simulink model "cable_driven_parallel_robot2022"  (R2022b)
settings: Solver=ode3  StartTime=0.0  StopTime=100  FixedStep=0.01  RelTol=1e-3
values from neighbouring files (symbols this model uses):
  cable_length = 1.2    [Model_Info.m]
  g = 9.81    [Model_Info.m]
  MP_H = 2    [Model_Info.m]
  MP_init_X = 0    [Model_Info.m]
  MP_init_Y = 0    [Model_Info.m]
  MP_init_Z = cable_length + (MP_H/2)    (= 2.2)    [Model_Info.m]
  MP_Ix = (MP_m/12)*(MP_W^2+MP_H^2)    (= 6.66666666667e-05)    [Model_Info.m]
  MP_Iy = (MP_m/12)*(MP_L^2+MP_H^2)    (= 6.66666666667e-05)    [Model_Info.m]
  MP_Iz = (MP_m/12)*(MP_L^2+MP_W^2)    (= 6.66666666667e-05)    [Model_Info.m]
  MP_L = 2    [Model_Info.m]
  MP_m = 0.0001    [Model_Info.m]
  MP_W = 2    [Model_Info.m]
  MR_init_X_L1 = -(MP_L/2)    (= -1)    [Model_Info.m]
  MR_init_X_L2 = (MP_L/2)    (= 1)    [Model_Info.m]
  MR_init_X_L3 = (MP_L/2)    (= 1)    [Model_Info.m]
  MR_init_X_L4 = -(MP_L/2)    (= -1)    [Model_Info.m]
  MR_init_Y_L1 = -(MP_W/2)    (= -1)    [Model_Info.m]
  MR_init_Y_L2 = -(MP_W/2)    (= -1)    [Model_Info.m]
  MR_init_Y_L3 = (MP_W/2)    (= 1)    [Model_Info.m]
  MR_init_Y_L4 = (MP_W/2)    (= 1)    [Model_Info.m]
  MR_init_Yaw_L1 = pi    (= 3.14159265359)    [Model_Info.m]
  MR_init_Yaw_L2 = 0    [Model_Info.m]
  MR_init_Yaw_L3 = 0    [Model_Info.m]
  MR_init_Yaw_L4 = pi    (= 3.14159265359)    [Model_Info.m]
  MR_Jr = (MR_m/12)*(MR_L^2+MR_W^2)    (= 0.333333333333)    [Model_Info.m]
  MR_m = 0.5    [Model_Info.m]
  MR_r = 2    [Model_Info.m]
  MR_WT = 2    [Model_Info.m]
  QR_Ax = 0.25*0    (= 0)    [Model_Info.m]
  QR_Ay = 0.25*0    (= 0)    [Model_Info.m]
  QR_Az = 0.25*0    (= 0)    [Model_Info.m]
  QR_b = 1.14*1e-7    (= 1.14e-07)    [Model_Info.m]
  QR_Ixx = 4.856*1e-3    (= 0.004856)    [Model_Info.m]
  QR_Iyy = 4.856*1e-3    (= 0.004856)    [Model_Info.m]
  QR_Izz = 8.801*1e-3    (= 0.008801)    [Model_Info.m]
  QR_K = 2.980*1e-6    (= 2.98e-06)    [Model_Info.m]
  QR_l = 0.225    [Model_Info.m]
  QR_m = 0.468    [Model_Info.m]
  QR_x0_U1 = -(MP_L/2)    (= -1)    [Model_Info.m]
  QR_x0_U2 = (MP_L/2)    (= 1)    [Model_Info.m]
  QR_x0_U3 = (MP_L/2)    (= 1)    [Model_Info.m]
  QR_x0_U4 = -(MP_L/2)    (= -1)    [Model_Info.m]
  QR_y0_U1 = -(MP_W/2)    (= -1)    [Model_Info.m]
  QR_y0_U2 = -(MP_W/2)    (= -1)    [Model_Info.m]
  QR_y0_U3 = (MP_W/2)    (= 1)    [Model_Info.m]
  QR_y0_U4 = (MP_W/2)    (= 1)    [Model_Info.m]
  QR_z0_U1 = 2*cable_length+(MP_H)    (= 4.4)    [Model_Info.m]
  QR_z0_U2 = 2*cable_length+(MP_H)    (= 4.4)    [Model_Info.m]
  QR_z0_U3 = 2*cable_length+(MP_H)    (= 4.4)    [Model_Info.m]
  QR_z0_U4 = 2*cable_length+(MP_H)    (= 4.4)    [Model_Info.m]
(part 6 of 12)

== matlab function cable_driven_parallel_robot2022/Actuators-CableTension-MovingPlatform/QuadRotor1/Subsystem/QuadCopter Model ==
  data: vx input; x_ddot output size=1; vy input; vz input; phidot input; thetadot input; psidot input; y_ddot output size=1; z_ddot output size=1; phi_ddot output size=1; theta_ddot output size=1; psi_ddot output size=1; phi input; theta input; psi input; constants input; z input; rest output
function [x_ddot,y_ddot,z_ddot,phi_ddot,theta_ddot,psi_ddot,rest] = fcn(vx,vy,vz,phidot,thetadot,psidot, phi,theta,psi,constants,z)
rest=0;
m = constants(1);
g = constants(2);
Ixx = constants(3);
Iyy = constants(4);
Izz = constants(5);
l = constants(6);
K = constants(7);
b = constants(8);
Ax = constants(9);
Ay = constants(10);
Az = constants(11);
omega1 = constants(12);
omega2 = constants(13);
omega3 = constants(14);
omega4 = constants(15);
Tx = constants(16);
Ty = constants(17);
Tz = constants(18);
% x_ddot = (K*omega1^2*sin(phi)*sin(psi) - Ax*vx + K*omega2^2*sin(phi)*sin(psi) + K*omega3^2*sin(phi)*sin(psi) + K*omega4^2*sin(phi)*sin(psi) + K*omega1^2*cos(phi)*cos(psi)*sin(theta) + K*omega2^2*cos(phi)*cos(psi)*sin(theta) + K*omega3^2*cos(phi)*cos(psi)*sin(theta) + K*omega4^2*cos(phi)*cos(psi)*sin(theta))/m;
% y_ddot = -(Ay*vy + K*omega1^2*cos(psi)*sin(phi) + K*omega2^2*cos(psi)*sin(phi) + K*omega3^2*cos(psi)*sin(phi) + K*omega4^2*cos(psi)*sin(phi) - K*omega1^2*cos(phi)*sin(psi)*sin(theta) - K*omega2^2*cos(phi)*sin(psi)*sin(theta) - K*omega3^2*cos(phi)*sin(psi)*sin(theta) - K*omega4^2*cos(phi)*sin(psi)*sin(theta))/m;
% z_ddot = (K*cos(phi)*cos(theta)*omega1^2 + K*cos(phi)*cos(theta)*omega2^2 + K*cos(phi)*cos(theta)*omega3^2 + K*cos(phi)*cos(theta)*omega4^2 - Az*vz - g*m)/m;
% phi_ddot = (2*Ixx*Iyy*b*omega1^2*sin(theta) - 2*Ixx*Iyy*b*omega2^2*sin(theta) + 2*Ixx*Iyy*b*omega3^2*sin(theta) - 2*Ixx*Iyy*b*omega4^2*sin(theta) + 2*Iyy^3*psidot^2*cos(phi)*cos(theta)^4*sin(phi)^3 - 2*Iyy^3*psidot^2*cos(phi)*cos(theta)^4*sin(phi)^5 - 2*Iyy^3*psidot*thetadot*cos(theta)^3*sin(phi)^2 + 2*Iyy^3*psidot*thetadot*cos(theta)^3*sin(phi)^4 - 2*Iyy^3*psidot^2*cos(phi)^3*cos(theta)^4*sin(phi)^3 - Iyy^3*thetadot^2*sin(2*phi)*cos(theta)^2*sin(phi)^2 + Iyy^3*thetadot^2*sin(2*phi)*cos(theta)^2*sin(phi)^4 - Ixx*Iyy^2*thetadot^2*sin(2*phi)*sin(theta)^2 - 2*Iyy^2*K*l*omega2^2*cos(theta)^2*sin(phi)^2 + 2*Iyy^2*K*l*omega2^2*cos(theta)^2*sin(phi)^4 + 2*Iyy^2*K*l*omega4^2*cos(theta)^2*sin(phi)^2 - 2*Iyy^2*K*l*omega4^2*cos(theta)^2*sin(phi)^4 + 2*Ixx*Iyy^2*thetadot^2*cos(phi)*sin(phi)*sin(theta)^2 - 2*Ixx*Iyy*b*omega1^2*sin(phi)^2*sin(theta) + 2*Ixx*Iyy*b*omega2^2*sin(phi)^2*sin(theta) - 2*Ixx*Iyy*b*omega3^2*sin(phi)^2*sin(theta) + 2*Ixx*Iyy*b*omega4^2*sin(phi)^2*sin(theta) + 2*Ixx*Izz*b*omega1^2*sin(phi)^2*sin(theta) - 2*Ixx*Izz*b*omega2^2*sin(phi)^2*sin(theta) + 2*Ixx*Izz*b*omega3^2*sin(phi)^2*sin(theta) - 2*Ixx*Izz*b*omega4^2*sin(phi)^2*sin(theta) - 2*Ixx*Iyy^2*psidot*thetadot*cos(theta)*sin(theta)^2 + 2*Ixx^2*Iyy*psidot*thetadot*cos(theta)*sin(theta)^2 + 2*Ixx*Iyy^2*psidot*thetadot*sin(2*theta)*sin(theta) - 2*Ixx^2*Iyy*psidot*thetadot*sin(2*theta)*sin(theta) - 2*Iyy*Izz^2*psidot^2*cos(phi)^3*cos(theta)^4*sin(phi) - 2*Iyy^2*Izz*psidot^2*cos(phi)*cos(theta)^4*sin(phi)^3 + 2*Iyy^2*Izz*psidot^2*cos(phi)^3*cos(theta)^4*sin(phi) - 2*Iyy*Izz^2*psidot^2*cos(phi)*cos(theta)^4*sin(phi)^5 + 4*Iyy^2*Izz*psidot^2*cos(phi)*cos(theta)^4*sin(phi)^5 - 2*Ixx*Iyy^2*thetadot^2*cos(phi)*sin(phi)^3*sin(theta)^2 - 2*Ixx*Izz^2*thetadot^2*cos(phi)*sin(phi)^3*sin(theta)^2 + Ixx*Iyy*Izz*thetadot^2*sin(2*phi)*sin(theta)^2 + 6*Iyy^3*psidot*thetadot*cos(phi)^2*cos(theta)^3*sin(phi)^2 - 4*Iyy^3*psidot*thetadot*cos(phi)^2*cos(theta)^3*sin(phi)^4 - 4*Iyy^3*psidot*thetadot*cos(phi)^4*cos(theta)^3*sin(phi)^2 + 2*Iyy*Izz^2*psidot*thetadot*cos(phi)^2*cos(theta)^3 - 2*Iyy^2*Izz*psidot*thetadot*cos(phi)^2*cos(theta)^3 - 4*Iyy*Izz^2*psidot*thetadot*cos(phi)^4*cos(theta)^3 + 4*Iyy^2*Izz*psidot*thetadot*cos(phi)^4*cos(theta)^3 + 2*Ixx*Iyy^2*psidot*thetadot*cos(theta)^3*sin(phi)^2 - 2*Ixx*Iyy^2*psidot*thetadot*cos(theta)^3*sin(phi)^4 + 2*Iyy^2*Izz*psidot*thetadot*cos(theta)^3*sin(phi)^2 + 2*Iyy*Izz^2*psidot*thetadot*cos(theta)^3*sin(phi)^4 - 4*Iyy^2*Izz*psidot*thetadot*cos(theta)^3*sin(phi)^4 - 2*Ixx*Iyy*K*l*omega2^2*sin(theta)^2 + 2*Ixx*Iyy*K*l*omega4^2*sin(theta)^2 + Iyy^3*thetadot^2*sin(2*phi)*cos(phi)^2*cos(theta)^2*sin(phi)^2 - 2*Iyy*Izz^2*psidot^2*cos(phi)^3*cos(theta)^4*sin(phi)^3 + 4*Iyy^2*Izz*psidot^2*cos(phi)^3*cos(theta)^4*sin(phi)^3 + Iyy*Izz^2*thetadot^2*sin(2*phi)*cos(phi)^2*cos(theta)^2 - Iyy^2*Izz*thetadot^2*sin(2*phi)*cos(phi)^2*cos(theta)^2 + Iyy^2*Izz*thetadot^2*sin(2*phi)*cos(theta)^2*sin(phi)^2 + Iyy*Izz^2*thetadot^2*sin(2*phi)*cos(theta)^2*sin(phi)^4 - 2*Iyy^2*Izz*thetadot^2*sin(2*phi)*cos(theta)^2*sin(phi)^4 + Ixx*Iyy^2*thetadot^2*sin(2*phi)*sin(phi)^2*sin(theta)^2 + Ixx*Izz^2*thetadot^2*sin(2*phi)*sin(phi)^2*sin(theta)^2 + 2*Ixx*Iyy^2*phidot*thetadot*cos(theta)*sin(theta) + 2*Ixx^2*Iyy*phidot*thetadot*cos(theta)*sin(theta) + 2*Ixx*Iyy*K*l*omega2^2*sin(phi)^2*sin(theta)^2 - 2*Ixx*Iyy*K*l*omega4^2*sin(phi)^2*sin(theta)^2 - 2*Ixx*Izz*K*l*omega2^2*sin(phi)^2*sin(theta)^2 + 2*Ixx*Izz*K*l*omega4^2*sin(phi)^2*sin(theta)^2 - 2*Ixx*Iyy*Izz*thetadot^2*cos(phi)*sin(phi)*sin(theta)^2 + Iyy*Izz^2*thetadot^2*sin(2*phi)*cos(phi)^2*cos(theta)^2*sin(phi)^2 - 2*Iyy^2*Izz*thetadot^2*sin(2*phi)*cos(phi)^2*cos(theta)^2*sin(phi)^2 - 4*Ixx*Iyy^2*phidot*thetadot*cos(phi)^2*cos(theta)*sin(theta) - 2*Ixx*Iyy^2*phidot*thetadot*cos(theta)*sin(phi)^2*sin(theta) - 2*Ixx^2*Iyy*phidot*thetadot*cos(theta)*sin(phi)^2*sin(theta) - 2*Ixx*Izz^2*phidot*thetadot*cos(theta)*sin(phi)^2*sin(theta) + 2*Ixx^2*Izz*phidot*thetadot*cos(theta)*sin(phi)^2*sin(theta) + 2*Iyy^2*K*l*omega2^2*cos(phi)^2*cos(theta)^2*sin(phi)^2 - 2*Iyy^2*K*l*omega4^2*cos(phi)^2*cos(theta)^2*sin(phi)^2 + 2*Ixx*Iyy*Izz*psidot*thetadot*cos(theta)*sin(theta)^2 + 2*Ixx*Iyy^2*psidot^2*cos(phi)*cos(theta)^2*sin(phi)*sin(theta)^2 + 4*Ixx*Iyy*Izz*thetadot^2*cos(phi)*sin(phi)^3*sin(theta)^2 + 2*Ixx*Iyy*Izz*psidot*thetadot*cos(phi)^2*cos(theta)^3 + 2*Ixx*Iyy^2*psidot*thetadot*cos(theta)*sin(phi)^2*sin(theta)^2 - 2*Ixx^2*Iyy*psidot*thetadot*cos(theta)*sin(phi)^2*sin(theta)^2 + 2*Ixx*Izz^2*psidot*thetadot*cos(theta)*sin(phi)^2*sin(theta)^2 + 2*Ixx^2*Izz*psidot*thetadot*cos(theta)*sin(phi)^2*sin(theta)^2 + 2*Ixx*Iyy*Izz*psidot*thetadot*cos(theta)^3*sin(phi)^4 - 2*Ixx*Iyy^2*psidot*thetadot*sin(2*theta)*sin(phi)^2*sin(theta) + 2*Ixx^2*Iyy*psidot*thetadot*sin(2*theta)*sin(phi)^2*sin(theta) - 2*Ixx^2*Izz*psidot*thetadot*sin(2*theta)*sin(phi)^2*sin(theta) - 2*Ixx*Izz^2*psidot^2*cos(phi)*cos(theta)^2*sin(phi)^3*sin(theta)^2 - 2*Ixx*Izz^2*psidot^2*cos(phi)^3*cos(theta)^2*sin(phi)*sin(theta)^2 - 2*Ixx*Iyy*Izz*thetadot^2*sin(2*phi)*sin(phi)^2*sin(theta)^2 - 2*Ixx*Iyy*Izz*phidot*thetadot*cos(theta)*sin(theta) - 2*Iyy*Izz*K*l*omega2^2*cos(phi)^2*cos(theta)^2 + 2*Iyy*Izz*K*l*omega4^2*cos(phi)^2*cos(theta)^2 - 2*Ixx*Iyy^2*psidot*thetadot*cos(phi)^2*cos(theta)^3*sin(phi)^2 + 2*Iyy*Izz^2*psidot*thetadot*cos(phi)^2*cos(theta)^3*sin(phi)^2 - 8*Iyy^2*Izz*psidot*thetadot*cos(phi)^2*cos(theta)^3*sin(phi)^2 - 4*Iyy*Izz^2*psidot*thetadot*cos(phi)^2*cos(theta)^3*sin(phi)^4 - 4*Iyy*Izz^2*psidot*thetadot*cos(phi)^4*cos(theta)^3*sin(phi)^2 + 8*Iyy^2*Izz*psidot*thetadot*cos(phi)^2*cos(theta)^3*sin(phi)^4 + 8*Iyy^2*Izz*psidot*thetadot*cos(phi)^4*cos(theta)^3*sin(phi)^2 - 2*Iyy*Izz*K*l*omega2^2*cos(theta)^2*sin(phi)^4 + 2*Iyy*Izz*K*l*omega4^2*cos(theta)^2*sin(phi)^4 - 4*Ixx*Iyy^2*phidot*psidot*cos(phi)*cos(theta)^2*sin(phi)*sin(theta) + 2*Ixx^2*Iyy*phidot*psidot*cos(phi)*cos(theta)^2*sin(phi)*sin(theta) - 2*Ixx^2*Izz*phidot*psidot*cos(phi)*cos(theta)^2*sin(phi)*sin(theta) + 4*Ixx*Iyy*Izz*phidot*thetadot*cos(phi)^2*cos(theta)*sin(theta) + 4*Ixx*Iyy*Izz*phidot*thetadot*cos(theta)*sin(phi)^2*sin(theta) - 2*Iyy*Izz*K*l*omega2^2*cos(phi)^2*cos(theta)^2*sin(phi)^2 + 2*Iyy*Izz*K*l*omega4^2*cos(phi)^2*cos(theta)^2*sin(phi)^2 - 2*Ixx*Iyy*Izz*psidot^2*cos(phi)*cos(theta)^2*sin(phi)*sin(theta)^2 + 2*Ixx*Iyy^2*phidot*psidot*cos(phi)*cos(theta)^2*sin(phi)^3*sin(theta) + 2*Ixx*Iyy^2*phidot*psidot*cos(phi)^3*cos(theta)^2*sin(phi)*sin(theta) + 2*Ixx*Izz^2*phidot*psidot*cos(phi)*cos(theta)^2*sin(phi)^3*sin(theta) + 2*Ixx*Izz^2*phidot*psidot*cos(phi)^3*cos(theta)^2*sin(phi)*sin(theta) + 4*Ixx*Iyy^2*phidot*thetadot*cos(phi)^2*cos(theta)*sin(phi)^2*sin(theta) + 4*Ixx*Izz^2*phidot*thetadot*cos(phi)^2*cos(theta)*sin(phi)^2*sin(theta) - 4*Ixx*Iyy*Izz*psidot*thetadot*cos(theta)*sin(phi)^2*sin(theta)^2 + 2*Ixx*Iyy*Izz*psidot*thetadot*sin(2*theta)*sin(phi)^2*sin(theta) + 2*Ixx*Iyy*Izz*psidot^2*cos(phi)*cos(theta)^2*sin(phi)^3*sin(theta)^2 + 2*Ixx*Iyy*Izz*psidot^2*cos(phi)^3*cos(theta)^2*sin(phi)*sin(theta)^2 + 2*Ixx*Iyy*Izz*psidot*thetadot*cos(phi)^2*cos(theta)^3*sin(phi)^2 - Ixx^2*Iyy*psidot^2*sin(2*theta)*cos(phi)*cos(theta)*sin(phi)*sin(theta) + Ixx^2*Izz*psidot^2*sin(2*theta)*cos(phi)*cos(theta)*sin(phi)*sin(theta) - 4*Ixx*Iyy*Izz*phidot*psidot*cos(phi)*cos(theta)^2*sin(phi)^3*sin(theta) - 4*Ixx*Iyy*Izz*phidot*psidot*cos(phi)^3*cos(theta)^2*sin(phi)*sin(theta) - 8*Ixx*Iyy*Izz*phidot*thetadot*cos(phi)^2*cos(theta)*sin(phi)^2*sin(theta) + 2*Ixx*Iyy*K*l*omega1^2*cos(phi)*cos(theta)*sin(phi)*sin(theta) - 2*Ixx*Iyy*K*l*omega3^2*cos(phi)*cos(theta)*sin(phi)*sin(theta) - 2*Ixx*Izz*K*l*omega1^2*cos(phi)*cos(theta)*sin(phi)*sin(theta) + 2*Ixx*Izz*K*l*omega3^2*cos(phi)*cos(theta)*sin(phi)*sin(theta) - 2*Ixx*Iyy^2*phidot*thetadot*sin(2*phi)*cos(phi)*cos(theta)*sin(phi)*sin(theta) - 2*Ixx*Izz^2*phidot*thetadot*sin(2*phi)*cos(phi)*cos(theta)*sin(phi)*sin(theta) + 4*Ixx*Iyy*Izz*phidot*psidot*cos(phi)*cos(theta)^2*sin(phi)*sin(theta) + 4*Ixx*Iyy*Izz*phidot*thetadot*sin(2*phi)*cos(phi)*cos(theta)*sin(phi)*sin(theta))/(2*Ixx*cos(theta)^2*(- Iyy^2*cos(phi)^2*sin(phi)^2 - Iyy^2*sin(phi)^4 + Iyy^2*sin(phi)^2 + Izz*Iyy*cos(phi)^2*sin(phi)^2 + Izz*Iyy*cos(phi)^2 + Izz*Iyy*sin(phi)^4));
% theta_ddot = -(2*Izz^2*psidot^2*cos(phi)^4*cos(theta)^2*sin(theta) + 2*Iyy^2*thetadot^2*cos(phi)^2*sin(phi)^2*sin(theta) + 2*Izz^2*thetadot^2*cos(phi)^2*sin(phi)^2*sin(theta) + 2*Iyy^2*psidot^2*cos(theta)^2*sin(phi)^4*sin(theta) - 2*Izz^2*phidot*psidot*cos(phi)^4*cos(theta)^2 - 2*Iyy^2*phidot*psidot*cos(theta)^2*sin(phi)^4 + 2*Iyy*b*omega1^2*cos(phi)*sin(phi) - 2*Iyy*b*omega2^2*cos(phi)*sin(phi) + 2*Iyy*b*omega3^2*cos(phi)*sin(phi) - 2*Iyy*b*omega4^2*cos(phi)*sin(phi) - 2*Izz*b*omega1^2*cos(phi)*sin(phi) + 2*Izz*b*omega2^2*cos(phi)*sin(phi) - 2*Izz*b*omega3^2*cos(phi)*sin(phi) + 2*Izz*b*omega4^2*cos(phi)*sin(phi) - Ixx*Izz*psidot^2*sin(2*theta)*cos(phi)^2*cos(theta) - 4*Iyy*Izz*thetadot^2*cos(phi)^2*sin(phi)^2*sin(theta) - Ixx*Iyy*psidot^2*sin(2*theta)*cos(theta)*sin(phi)^2 + 2*Izz*K*l*omega1^2*cos(phi)^2*cos(theta) - 2*Izz*K*l*omega3^2*cos(phi)^2*cos(theta) + 2*Izz^2*phidot*thetadot*sin(2*phi)*cos(phi)^2*cos(theta) + 2*Ixx*Izz*phidot*psidot*cos(phi)^2*cos(theta)^2 + 2*Iyy*Izz*phidot*psidot*cos(phi)^4*cos(theta)^2 + 2*Iyy*K*l*omega1^2*cos(theta)*sin(phi)^2 - 2*Iyy*K*l*omega3^2*cos(theta)*sin(phi)^2 - 2*Iyy^2*phidot*thetadot*sin(2*phi)*cos(theta)*sin(phi)^2 + 2*Ixx*Iyy*phidot*psidot*cos(theta)^2*sin(phi)^2 + 2*Iyy*Izz*phidot*psidot*cos(theta)^2*sin(phi)^4 + 2*Iyy^2*psidot^2*cos(phi)^2*cos(theta)^2*sin(phi)^2*sin(theta) + 2*Izz^2*psidot^2*cos(phi)^2*cos(theta)^2*sin(phi)^2*sin(theta) + 2*Iyy^2*phidot*thetadot*cos(phi)*cos(theta)*sin(phi) + 2*Izz^2*phidot*thetadot*cos(phi)*cos(theta)*sin(phi) - 2*Iyy^2*phidot*psidot*cos(phi)^2*cos(theta)^2*sin(phi)^2 - 2*Izz^2*phidot*psidot*cos(phi)^2*cos(theta)^2*sin(phi)^2 - Iyy^2*thetadot^2*sin(2*phi)*cos(phi)*sin(phi)*sin(theta) - Izz^2*thetadot^2*sin(2*phi)*cos(phi)*sin(phi)*sin(theta) - 4*Iyy^2*phidot*thetadot*cos(phi)^3*cos(theta)*sin(phi) - 4*Izz^2*phidot*thetadot*cos(phi)^3*cos(theta)*sin(phi) + 2*Iyy^2*psidot*thetadot*sin(2*theta)*cos(phi)*sin(phi) - 2*Iyy*Izz*phidot*thetadot*sin(2*phi)*cos(phi)^2*cos(theta) + 2*Iyy*Izz*phidot*thetadot*sin(2*phi)*cos(theta)*sin(phi)^2 - 2*Iyy^2*psidot*thetadot*cos(phi)*cos(theta)*sin(phi)*sin(theta) - 2*Izz^2*psidot*thetadot*cos(phi)*cos(theta)*sin(phi)*sin(theta) + 2*Ixx*Iyy*phidot*thetadot*cos(phi)*cos(theta)*sin(phi) - 2*Ixx*Izz*phidot*thetadot*cos(phi)*cos(theta)*sin(phi) - 4*Iyy*Izz*phidot*thetadot*cos(phi)*cos(theta)*sin(phi) + 4*Iyy*Izz*phidot*psidot*cos(phi)^2*cos(theta)^2*sin(phi)^2 + 2*Iyy*Izz*thetadot^2*sin(2*phi)*cos(phi)*sin(phi)*sin(theta) + 8*Iyy*Izz*phidot*thetadot*cos(phi)^3*cos(theta)*sin(phi) - 2*Iyy*K*l*omega2^2*cos(phi)*sin(phi)*sin(theta) + 2*Iyy*K*l*omega4^2*cos(phi)*sin(phi)*sin(theta) + 2*Izz*K*l*omega2^2*cos(phi)*sin(phi)*sin(theta) - 2*Izz*K*l*omega4^2*cos(phi)*sin(phi)*sin(theta) - 2*Ixx*Iyy*psidot*thetadot*sin(2*theta)*cos(phi)*sin(phi) + 2*Ixx*Izz*psidot*thetadot*sin(2*theta)*cos(phi)*sin(phi) - 2*Iyy*Izz*psidot*thetadot*sin(2*theta)*cos(phi)*sin(phi) + 2*Ixx*Iyy*psidot*thetadot*cos(phi)*cos(theta)*sin(phi)*sin(theta) - 2*Ixx*Izz*psidot*thetadot*cos(phi)*cos(theta)*sin(phi)*sin(theta) + 4*Iyy*Izz*psidot*thetadot*cos(phi)*cos(theta)*sin(phi)*sin(theta))/(2*cos(theta)*(- Iyy^2*cos(phi)^2*sin(phi)^2 - Iyy^2*sin(phi)^4 + Iyy^2*sin(phi)^2 + Izz*Iyy*cos(phi)^2*sin(phi)^2 + Izz*Iyy*cos(phi)^2 + Izz*Iyy*sin(phi)^4));
% psi_ddot = (2*Iyy*b*omega1^2 - 2*Iyy*b*omega2^2 + 2*Iyy*b*omega3^2 - 2*Iyy*b*omega4^2 - Iyy^2*thetadot^2*sin(2*phi)*sin(theta) - 2*Iyy*b*omega1^2*sin(phi)^2 + 2*Iyy*b*omega2^2*sin(phi)^2 - 2*Iyy*b*omega3^2*sin(phi)^2 + 2*Iyy*b*omega4^2*sin(phi)^2 + 2*Izz*b*omega1^2*sin(phi)^2 - 2*Izz*b*omega2^2*sin(phi)^2 + 2*Izz*b*omega3^2*sin(phi)^2 - 2*Izz*b*omega4^2*sin(phi)^2 + 2*Iyy^2*psidot*thetadot*sin(2*theta) + 2*Iyy^2*phidot*thetadot*cos(theta) - 2*Iyy^2*phidot*thetadot*cos(theta)*sin(phi)^2 - 2*Izz^2*phidot*thetadot*cos(theta)*sin(phi)^2 - 2*Iyy*K*l*omega2^2*sin(theta) + 2*Iyy*K*l*omega4^2*sin(theta) - 2*Ixx*Iyy*psidot*thetadot*sin(2*theta) + Iyy^2*thetadot^2*sin(2*phi)*sin(phi)^2*sin(theta) + Izz^2*thetadot^2*sin(2*phi)*sin(phi)^2*sin(theta) - 2*Iyy^2*psidot*thetadot*sin(2*theta)*sin(phi)^2 + 2*Iyy^2*thetadot^2*cos(phi)*sin(phi)*sin(theta) - 2*Iyy^2*psidot*thetadot*cos(theta)*sin(theta) + 2*Ixx*Iyy*phidot*thetadot*cos(theta) - 2*Iyy*Izz*phidot*thetadot*cos(theta) - 2*Iyy^2*thetadot^2*cos(phi)*sin(phi)^3*sin(theta) - 2*Izz^2*thetadot^2*cos(phi)*sin(phi)^3*sin(theta) + Iyy*Izz*thetadot^2*sin(2*phi)*sin(theta) - 4*Iyy^2*phidot*thetadot*cos(phi)^2*cos(theta) - 2*Izz^2*psidot^2*cos(phi)*cos(theta)^2*sin(phi)^3*sin(theta) - 2*Izz^2*psidot^2*cos(phi)^3*cos(theta)^2*sin(phi)*sin(theta) - 2*Iyy*Izz*thetadot^2*sin(2*phi)*sin(phi)^2*sin(theta) + 2*Iyy^2*phidot*psidot*cos(phi)*cos(theta)^2*sin(phi)^3 + 2*Iyy^2*phidot*psidot*cos(phi)^3*cos(theta)^2*sin(phi) + 2*Izz^2*phidot*psidot*cos(phi)*cos(theta)^2*sin(phi)^3 + 2*Izz^2*phidot*psidot*cos(phi)^3*cos(theta)^2*sin(phi) + 4*Iyy^2*phidot*thetadot*cos(phi)^2*cos(theta)*sin(phi)^2 + 4*Izz^2*phidot*thetadot*cos(phi)^2*cos(theta)*sin(phi)^2 + 2*Iyy*K*l*omega2^2*sin(phi)^2*sin(theta) - 2*Iyy*K*l*omega4^2*sin(phi)^2*sin(theta) - 2*Izz*K*l*omega2^2*sin(phi)^2*sin(theta) + 2*Izz*K*l*omega4^2*sin(phi)^2*sin(theta) + 2*Ixx*Iyy*psidot*thetadot*sin(2*theta)*sin(phi)^2 - 2*Ixx*Izz*psidot*thetadot*sin(2*theta)*sin(phi)^2 + 2*Iyy*Izz*psidot*thetadot*sin(2*theta)*sin(phi)^2 - 2*Iyy*Izz*thetadot^2*cos(phi)*sin(phi)*sin(theta) + 2*Ixx*Iyy*psidot*thetadot*cos(theta)*sin(theta) + 2*Iyy*Izz*psidot*thetadot*cos(theta)*sin(theta) + 2*Iyy^2*psidot^2*cos(phi)*cos(theta)^2*sin(phi)*sin(theta) + 4*Iyy*Izz*thetadot^2*cos(phi)*sin(phi)^3*sin(theta) - 4*Iyy^2*phidot*psidot*cos(phi)*cos(theta)^2*sin(phi) + 4*Iyy*Izz*phidot*thetadot*cos(phi)^2*cos(theta) + 2*Iyy^2*psidot*thetadot*cos(theta)*sin(phi)^2*sin(theta) + 2*Izz^2*psidot*thetadot*cos(theta)*sin(phi)^2*sin(theta) - 2*Ixx*Iyy*phidot*thetadot*cos(theta)*sin(phi)^2 + 2*Ixx*Izz*phidot*thetadot*cos(theta)*sin(phi)^2 + 4*Iyy*Izz*phidot*thetadot*cos(theta)*sin(phi)^2 - 4*Iyy*Izz*phidot*psidot*cos(phi)*cos(theta)^2*sin(phi)^3 - 4*Iyy*Izz*phidot*psidot*cos(phi)^3*cos(theta)^2*sin(phi) - 8*Iyy*Izz*phidot*thetadot*cos(phi)^2*cos(theta)*sin(phi)^2 - Ixx*Iyy*psidot^2*sin(2*theta)*cos(phi)*cos(theta)*sin(phi) + Ixx*Izz*psidot^2*sin(2*theta)*cos(phi)*cos(theta)*sin(phi) - 2*Iyy*Izz*psidot^2*cos(phi)*cos(theta)^2*sin(phi)*sin(theta) + 2*Iyy*K*l*omega1^2*cos(phi)*cos(theta)*sin(phi) - 2*Iyy*K*l*omega3^2*cos(phi)*cos(theta)*sin(phi) - 2*Izz*K*l*omega1^2*cos(phi)*cos(theta)*sin(phi) + 2*Izz*K*l*omega3^2*cos(phi)*cos(theta)*sin(phi) - 2*Iyy^2*phidot*thetadot*sin(2*phi)*cos(phi)*cos(theta)*sin(phi) - 2*Izz^2*phidot*thetadot*sin(2*phi)*cos(phi)*cos(theta)*sin(phi) + 2*Ixx*Iyy*phidot*psidot*cos(phi)*cos(theta)^2*sin(phi) - 2*Ixx*Izz*phidot*psidot*cos(phi)*cos(theta)^2*sin(phi) + 4*Iyy*Izz*phidot*psidot*cos(phi)*cos(theta)^2*sin(phi) - 2*Ixx*Iyy*psidot*thetadot*cos(theta)*sin(phi)^2*sin(theta) + 2*Ixx*Izz*psidot*thetadot*cos(theta)*sin(phi)^2*sin(theta) - 4*Iyy*Izz*psidot*thetadot*cos(theta)*sin(phi)^2*sin(theta) + 2*Iyy*Izz*psidot^2*cos(phi)*cos(theta)^2*sin(phi)^3*sin(theta) + 2*Iyy*Izz*psidot^2*cos(phi)^3*cos(theta)^2*sin(phi)*sin(theta) + 4*Iyy*Izz*phidot*thetadot*sin(2*phi)*cos(phi)*cos(theta)*sin(phi))/(2*cos(theta)^2*(- Iyy^2*cos(phi)^2*sin(phi)^2 - Iyy^2*sin(phi)^4 + Iyy^2*sin(phi)^2 + Izz*Iyy*cos(phi)^2*sin(phi)^2 + Izz*Iyy*cos(phi)^2 + Izz*Iyy*sin(phi)^4));
x_ddot =  (K*omega1^2*sin(phi)*sin(psi) - Ax*vx + Tx + K*omega2^2*sin(phi)*sin(psi) + K*omega3^2*sin(phi)*sin(psi) + K*omega4^2*sin(phi)*sin(psi) + K*omega1^2*cos(phi)*cos(psi)*sin(theta) + K*omega2^2*cos(phi)*cos(psi)*sin(theta) + K*omega3^2*cos(phi)*cos(psi)*sin(theta) + K*omega4^2*cos(phi)*cos(psi)*sin(theta))/m;
y_ddot = -(-Ty + Ay*vy + K*omega1^2*cos(psi)*sin(phi) + K*omega2^2*cos(psi)*sin(phi) + K*omega3^2*cos(psi)*sin(phi) + K*omega4^2*cos(psi)*sin(phi) - K*omega1^2*cos(phi)*sin(psi)*sin(theta) - K*omega2^2*cos(phi)*sin(psi)*sin(theta) - K*omega3^2*cos(phi)*sin(psi)*sin(theta) - K*omega4^2*cos(phi)*sin(psi)*sin(theta))/m;
z_ddot = (K*cos(phi)*cos(theta)*omega1^2 + K*cos(phi)*cos(theta)*omega2^2 + K*cos(phi)*cos(theta)*omega3^2 + K*cos(phi)*cos(theta)*omega4^2 + Tz - Az*vz - g*m)/m;
phi_ddot = (2*Ixx*Iyy*b*omega1^2*sin(theta) - 2*Ixx*Iyy*b*omega2^2*sin(theta) + 2*Ixx*Iyy*b*omega3^2*sin(theta) - 2*Ixx*Iyy*b*omega4^2*sin(theta) + 2*Iyy^3*psidot^2*cos(phi)*cos(theta)^4*sin(phi)^3 - 2*Iyy^3*psidot^2*cos(phi)*cos(theta)^4*sin(phi)^5 - 2*Iyy^3*psidot*thetadot*cos(theta)^3*sin(phi)^2 + 2*Iyy^3*psidot*thetadot*cos(theta)^3*sin(phi)^4 - 2*Iyy^3*psidot^2*cos(phi)^3*cos(theta)^4*sin(phi)^3 - Iyy^3*thetadot^2*sin(2*phi)*cos(theta)^2*sin(phi)^2 + Iyy^3*thetadot^2*sin(2*phi)*cos(theta)^2*sin(phi)^4 - Ixx*Iyy^2*thetadot^2*sin(2*phi)*sin(theta)^2 - 2*Iyy^2*K*l*omega2^2*cos(theta)^2*sin(phi)^2 + 2*Iyy^2*K*l*omega2^2*cos(theta)^2*sin(phi)^4 + 2*Iyy^2*K*l*omega4^2*cos(theta)^2*sin(phi)^2 - 2*Iyy^2*K*l*omega4^2*cos(theta)^2*sin(phi)^4 + 2*Ixx*Iyy^2*thetadot^2*cos(phi)*sin(phi)*sin(theta)^2 - 2*Ixx*Iyy*b*omega1^2*sin(phi)^2*sin(theta) + 2*Ixx*Iyy*b*omega2^2*sin(phi)^2*sin(theta) - 2*Ixx*Iyy*b*omega3^2*sin(phi)^2*sin(theta) + 2*Ixx*Iyy*b*omega4^2*sin(phi)^2*sin(theta) + 2*Ixx*Izz*b*omega1^2*sin(phi)^2*sin(theta) - 2*Ixx*Izz*b*omega2^2*sin(phi)^2*sin(theta) + 2*Ixx*Izz*b*omega3^2*sin(phi)^2*sin(theta) - 2*Ixx*Izz*b*omega4^2*sin(phi)^2*sin(theta) - 2*Ixx*Iyy^2*psidot*thetadot*cos(theta)*sin(theta)^2 + 2*Ixx^2*Iyy*psidot*thetadot*cos(theta)*sin(theta)^2 + 2*Ixx*Iyy^2*psidot*thetadot*sin(2*theta)*sin(theta) - 2*Ixx^2*Iyy*psidot*thetadot*sin(2*theta)*sin(theta) - 2*Iyy*Izz^2*psidot^2*cos(phi)^3*cos(theta)^4*sin(phi) - 2*Iyy^2*Izz*psidot^2*cos(phi)*cos(theta)^4*sin(phi)^3 + 2*Iyy^2*Izz*psidot^2*cos(phi)^3*cos(theta)^4*sin(phi) - 2*Iyy*Izz^2*psidot^2*cos(phi)*cos(theta)^4*sin(phi)^5 + 4*Iyy^2*Izz*psidot^2*cos(phi)*cos(theta)^4*sin(phi)^5 - 2*Ixx*Iyy^2*thetadot^2*cos(phi)*sin(phi)^3*sin(theta)^2 - 2*Ixx*Izz^2*thetadot^2*cos(phi)*sin(phi)^3*sin(theta)^2 + Ixx*Iyy*Izz*thetadot^2*sin(2*phi)*sin(theta)^2 + 6*Iyy^3*psidot*thetadot*cos(phi)^2*cos(theta)^3*sin(phi)^2 - 4*Iyy^3*psidot*thetadot*cos(phi)^2*cos(theta)^3*sin(phi)^4 - 4*Iyy^3*psidot*thetadot*cos(phi)^4*cos(theta)^3*sin(phi)^2 + 2*Iyy*Izz^2*psidot*thetadot*cos(phi)^2*cos(theta)^3 - 2*Iyy^2*Izz*psidot*thetadot*cos(phi)^2*cos(theta)^3 - 4*Iyy*Izz^2*psidot*thetadot*cos(phi)^4*cos(theta)^3 + 4*Iyy^2*Izz*psidot*thetadot*cos(phi)^4*cos(theta)^3 + 2*Ixx*Iyy^2*psidot*thetadot*cos(theta)^3*sin(phi)^2 - 2*Ixx*Iyy^2*psidot*thetadot*cos(theta)^3*sin(phi)^4 + 2*Iyy^2*Izz*psidot*thetadot*cos(theta)^3*sin(phi)^2 + 2*Iyy*Izz^2*psidot*thetadot*cos(theta)^3*sin(phi)^4 - 4*Iyy^2*Izz*psidot*thetadot*cos(theta)^3*sin(phi)^4 - 2*Ixx*Iyy*K*l*omega2^2*sin(theta)^2 + 2*Ixx*Iyy*K*l*omega4^2*sin(theta)^2 + Iyy^3*thetadot^2*sin(2*phi)*cos(phi)^2*cos(theta)^2*sin(phi)^2 - 2*Iyy*Izz^2*psidot^2*cos(phi)^3*cos(theta)^4*sin(phi)^3 + 4*Iyy^2*Izz*psidot^2*cos(phi)^3*cos(theta)^4*sin(phi)^3 + Iyy*Izz^2*thetadot^2*sin(2*phi)*cos(phi)^2*cos(theta)^2 - Iyy^2*Izz*thetadot^2*sin(2*phi)*cos(phi)^2*cos(theta)^2 + Iyy^2*Izz*thetadot^2*sin(2*phi)*cos(theta)^2*sin(phi)^2 + Iyy*Izz^2*thetadot^2*sin(2*phi)*cos(theta)^2*sin(phi)^4 - 2*Iyy^2*Izz*thetadot^2*sin(2*phi)*cos(theta)^2*sin(phi)^4 + Ixx*Iyy^2*thetadot^2*sin(2*phi)*sin(phi)^2*sin(theta)^2 + Ixx*Izz^2*thetadot^2*sin(2*phi)*sin(phi)^2*sin(theta)^2 + 2*Ixx*Iyy^2*phidot*thetadot*cos(theta)*sin(theta) + 2*Ixx^2*Iyy*phidot*thetadot*cos(theta)*sin(theta) + 2*Ixx*Iyy*K*l*omega2^2*sin(phi)^2*sin(theta)^2 - 2*Ixx*Iyy*K*l*omega4^2*sin(phi)^2*sin(theta)^2 - 2*Ixx*Izz*K*l*omega2^2*sin(phi)^2*sin(theta)^2 + 2*Ixx*Izz*K*l*omega4^2*sin(phi)^2*sin(theta)^2 - 2*Ixx*Iyy*Izz*thetadot^2*cos(phi)*sin(phi)*sin(theta)^2 + Iyy*Izz^2*thetadot^2*sin(2*phi)*cos(phi)^2*cos(theta)^2*sin(phi)^2 - 2*Iyy^2*Izz*thetadot^2*sin(2*phi)*cos(phi)^2*cos(theta)^2*sin(phi)^2 - 4*Ixx*Iyy^2*phidot*thetadot*cos(phi)^2*cos(theta)*sin(theta) - 2*Ixx*Iyy^2*phidot*thetadot*cos(theta)*sin(phi)^2*sin(theta) - 2*Ixx^2*Iyy*phidot*thetadot*cos(theta)*sin(phi)^2*sin(theta) - 2*Ixx*Izz^2*phidot*thetadot*cos(theta)*sin(phi)^2*sin(theta) + 2*Ixx^2*Izz*phidot*thetadot*cos(theta)*sin(phi)^2*sin(theta) + 2*Iyy^2*K*l*omega2^2*cos(phi)^2*cos(theta)^2*sin(phi)^2 - 2*Iyy^2*K*l*omega4^2*cos(phi)^2*cos(theta)^2*sin(phi)^2 + 2*Ixx*Iyy*Izz*psidot*thetadot*cos(theta)*sin(theta)^2 + 2*Ixx*Iyy^2*psidot^2*cos(phi)*cos(theta)^2*sin(phi)*sin(theta)^2 + 4*Ixx*Iyy*Izz*thetadot^2*cos(phi)*sin(phi)^3*sin(theta)^2 + 2*Ixx*Iyy*Izz*psidot*thetadot*cos(phi)^2*cos(theta)^3 + 2*Ixx*Iyy^2*psidot*thetadot*cos(theta)*sin(phi)^2*sin(theta)^2 - 2*Ixx^2*Iyy*psidot*thetadot*cos(theta)*sin(phi)^2*sin(theta)^2 + 2*Ixx*Izz^2*psidot*thetadot*cos(theta)*sin(phi)^2*sin(theta)^2 + 2*Ixx^2*Izz*psidot*thetadot*cos(theta)*sin(phi)^2*sin(theta)^2 + 2*Ixx*Iyy*Izz*psidot*thetadot*cos(theta)^3*sin(phi)^4 - 2*Ixx*Iyy^2*psidot*thetadot*sin(2*theta)*sin(phi)^2*sin(theta) + 2*Ixx^2*Iyy*psidot*thetadot*sin(2*theta)*sin(phi)^2*sin(theta) - 2*Ixx^2*Izz*psidot*thetadot*sin(2*theta)*sin(phi)^2*sin(theta) - 2*Ixx*Izz^2*psidot^2*cos(phi)*cos(theta)^2*sin(phi)^3*sin(theta)^2 - 2*Ixx*Izz^2*psidot^2*cos(phi)^3*cos(theta)^2*sin(phi)*sin(theta)^2 - 2*Ixx*Iyy*Izz*thetadot^2*sin(2*phi)*sin(phi)^2*sin(theta)^2 - 2*Ixx*Iyy*Izz*phidot*thetadot*cos(theta)*sin(theta) - 2*Iyy*Izz*K*l*omega2^2*cos(phi)^2*cos(theta)^2 + 2*Iyy*Izz*K*l*omega4^2*cos(phi)^2*cos(theta)^2 - 2*Ixx*Iyy^2*psidot*thetadot*cos(phi)^2*cos(theta)^3*sin(phi)^2 + 2*Iyy*Izz^2*psidot*thetadot*cos(phi)^2*cos(theta)^3*sin(phi)^2 - 8*Iyy^2*Izz*psidot*thetadot*cos(phi)^2*cos(theta)^3*sin(phi)^2 - 4*Iyy*Izz^2*psidot*thetadot*cos(phi)^2*cos(theta)^3*sin(phi)^4 - 4*Iyy*Izz^2*psidot*thetadot*cos(phi)^4*cos(theta)^3*sin(phi)^2 + 8*Iyy^2*Izz*psidot*thetadot*cos(phi)^2*cos(theta)^3*sin(phi)^4 + 8*Iyy^2*Izz*psidot*thetadot*cos(phi)^4*cos(theta)^3*sin(phi)^2 - 2*Iyy*Izz*K*l*omega2^2*cos(theta)^2*sin(phi)^4 + 2*Iyy*Izz*K*l*omega4^2*cos(theta)^2*sin(phi)^4 - 4*Ixx*Iyy^2*phidot*psidot*cos(phi)*cos(theta)^2*sin(phi)*sin(theta) + 2*Ixx^2*Iyy*phidot*psidot*cos(phi)*cos(theta)^2*sin(phi)*sin(theta) - 2*Ixx^2*Izz*phidot*psidot*cos(phi)*cos(theta)^2*sin(phi)*sin(theta) + 4*Ixx*Iyy*Izz*phidot*thetadot*cos(phi)^2*cos(theta)*sin(theta) + 4*Ixx*Iyy*Izz*phidot*thetadot*cos(theta)*sin(phi)^2*sin(theta) - 2*Iyy*Izz*K*l*omega2^2*cos(phi)^2*cos(theta)^2*sin(phi)^2 + 2*Iyy*Izz*K*l*omega4^2*cos(phi)^2*cos(theta)^2*sin(phi)^2 - 2*Ixx*Iyy*Izz*psidot^2*cos(phi)*cos(theta)^2*sin(phi)*sin(theta)^2 + 2*Ixx*Iyy^2*phidot*psidot*cos(phi)*cos(theta)^2*sin(phi)^3*sin(theta) + 2*Ixx*Iyy^2*phidot*psidot*cos(phi)^3*cos(theta)^2*sin(phi)*sin(theta) + 2*Ixx*Izz^2*phidot*psidot*cos(phi)*cos(theta)^2*sin(phi)^3*sin(theta) + 2*Ixx*Izz^2*phidot*psidot*cos(phi)^3*cos(theta)^2*sin(phi)*sin(theta) + 4*Ixx*Iyy^2*phidot*thetadot*cos(phi)^2*cos(theta)*sin(phi)^2*sin(theta) + 4*Ixx*Izz^2*phidot*thetadot*cos(phi)^2*cos(theta)*sin(phi)^2*sin(theta) - 4*Ixx*Iyy*Izz*psidot*thetadot*cos(theta)*sin(phi)^2*sin(theta)^2 + 2*Ixx*Iyy*Izz*psidot*thetadot*sin(2*theta)*sin(phi)^2*sin(theta) + 2*Ixx*Iyy*Izz*psidot^2*cos(phi)*cos(theta)^2*sin(phi)^3*sin(theta)^2 + 2*Ixx*Iyy*Izz*psidot^2*cos(phi)^3*cos(theta)^2*sin(phi)*sin(theta)^2 + 2*Ixx*Iyy*Izz*psidot*thetadot*cos(phi)^2*cos(theta)^3*sin(phi)^2 - Ixx^2*Iyy*psidot^2*sin(2*theta)*cos(phi)*cos(theta)*sin(phi)*sin(theta) + Ixx^2*Izz*psidot^2*sin(2*theta)*cos(phi)*cos(theta)*sin(phi)*sin(theta) - 4*Ixx*Iyy*Izz*phidot*psidot*cos(phi)*cos(theta)^2*sin(phi)^3*sin(theta) - 4*Ixx*Iyy*Izz*phidot*psidot*cos(phi)^3*cos(theta)^2*sin(phi)*sin(theta) - 8*Ixx*Iyy*Izz*phidot*thetadot*cos(phi)^2*cos(theta)*sin(phi)^2*sin(theta) + 2*Ixx*Iyy*K*l*omega1^2*cos(phi)*cos(theta)*sin(phi)*sin(theta) - 2*Ixx*Iyy*K*l*omega3^2*cos(phi)*cos(theta)*sin(phi)*sin(theta) - 2*Ixx*Izz*K*l*omega1^2*cos(phi)*cos(theta)*sin(phi)*sin(theta) + 2*Ixx*Izz*K*l*omega3^2*cos(phi)*cos(theta)*sin(phi)*sin(theta) - 2*Ixx*Iyy^2*phidot*thetadot*sin(2*phi)*cos(phi)*cos(theta)*sin(phi)*sin(theta) - 2*Ixx*Izz^2*phidot*thetadot*sin(2*phi)*cos(phi)*cos(theta)*sin(phi)*sin(theta) + 4*Ixx*Iyy*Izz*phidot*psidot*cos(phi)*cos(theta)^2*sin(phi)*sin(theta) + 4*Ixx*Iyy*Izz*phidot*thetadot*sin(2*phi)*cos(phi)*cos(theta)*sin(phi)*sin(theta))/(2*Ixx*cos(theta)^2*(- Iyy^2*cos(phi)^2*sin(phi)^2 - Iyy^2*sin(phi)^4 + Iyy^2*sin(phi)^2 + Izz*Iyy*cos(phi)^2*sin(phi)^2 + Izz*Iyy*cos(phi)^2 + Izz*Iyy*sin(phi)^4));
theta_ddot = -(2*Izz^2*psidot^2*cos(phi)^4*cos(theta)^2*sin(theta) + 2*Iyy^2*thetadot^2*cos(phi)^2*sin(phi)^2*sin(theta) + 2*Izz^2*thetadot^2*cos(phi)^2*sin(phi)^2*sin(theta) + 2*Iyy^2*psidot^2*cos(theta)^2*sin(phi)^4*sin(theta) - 2*Izz^2*phidot*psidot*cos(phi)^4*cos(theta)^2 - 2*Iyy^2*phidot*psidot*cos(theta)^2*sin(phi)^4 + 2*Iyy*b*omega1^2*cos(phi)*sin(phi) - 2*Iyy*b*omega2^2*cos(phi)*sin(phi) + 2*Iyy*b*omega3^2*cos(phi)*sin(phi) - 2*Iyy*b*omega4^2*cos(phi)*sin(phi) - 2*Izz*b*omega1^2*cos(phi)*sin(phi) + 2*Izz*b*omega2^2*cos(phi)*sin(phi) - 2*Izz*b*omega3^2*cos(phi)*sin(phi) + 2*Izz*b*omega4^2*cos(phi)*sin(phi) - Ixx*Izz*psidot^2*sin(2*theta)*cos(phi)^2*cos(theta) - 4*Iyy*Izz*thetadot^2*cos(phi)^2*sin(phi)^2*sin(theta) - Ixx*Iyy*psidot^2*sin(2*theta)*cos(theta)*sin(phi)^2 + 2*Izz*K*l*omega1^2*cos(phi)^2*cos(theta) - 2*Izz*K*l*omega3^2*cos(phi)^2*cos(theta) + 2*Izz^2*phidot*thetadot*sin(2*phi)*cos(phi)^2*cos(theta) + 2*Ixx*Izz*phidot*psidot*cos(phi)^2*cos(theta)^2 + 2*Iyy*Izz*phidot*psidot*cos(phi)^4*cos(theta)^2 + 2*Iyy*K*l*omega1^2*cos(theta)*sin(phi)^2 - 2*Iyy*K*l*omega3^2*cos(theta)*sin(phi)^2 - 2*Iyy^2*phidot*thetadot*sin(2*phi)*cos(theta)*sin(phi)^2 + 2*Ixx*Iyy*phidot*psidot*cos(theta)^2*sin(phi)^2 + 2*Iyy*Izz*phidot*psidot*cos(theta)^2*sin(phi)^4 + 2*Iyy^2*psidot^2*cos(phi)^2*cos(theta)^2*sin(phi)^2*sin(theta) + 2*Izz^2*psidot^2*cos(phi)^2*cos(theta)^2*sin(phi)^2*sin(theta) + 2*Iyy^2*phidot*thetadot*cos(phi)*cos(theta)*sin(phi) + 2*Izz^2*phidot*thetadot*cos(phi)*cos(theta)*sin(phi) - 2*Iyy^2*phidot*psidot*cos(phi)^2*cos(theta)^2*sin(phi)^2 - 2*Izz^2*phidot*psidot*cos(phi)^2*cos(theta)^2*sin(phi)^2 - Iyy^2*thetadot^2*sin(2*phi)*cos(phi)*sin(phi)*sin(theta) - Izz^2*thetadot^2*sin(2*phi)*cos(phi)*sin(phi)*sin(theta) - 4*Iyy^2*phidot*thetadot*cos(phi)^3*cos(theta)*sin(phi) - 4*Izz^2*phidot*thetadot*cos(phi)^3*cos(theta)*sin(phi) + 2*Iyy^2*psidot*thetadot*sin(2*theta)*cos(phi)*sin(phi) - 2*Iyy*Izz*phidot*thetadot*sin(2*phi)*cos(phi)^2*cos(theta) + 2*Iyy*Izz*phidot*thetadot*sin(2*phi)*cos(theta)*sin(phi)^2 - 2*Iyy^2*psidot*thetadot*cos(phi)*cos(theta)*sin(phi)*sin(theta) - 2*Izz^2*psidot*thetadot*cos(phi)*cos(theta)*sin(phi)*sin(theta) + 2*Ixx*Iyy*phidot*thetadot*cos(phi)*cos(theta)*sin(phi) - 2*Ixx*Izz*phidot*thetadot*cos(phi)*cos(theta)*sin(phi) - 4*Iyy*Izz*phidot*thetadot*cos(phi)*cos(theta)*sin(phi) + 4*Iyy*Izz*phidot*psidot*cos(phi)^2*cos(theta)^2*sin(phi)^2 + 2*Iyy*Izz*thetadot^2*sin(2*phi)*cos(phi)*sin(phi)*sin(theta) + 8*Iyy*Izz*phidot*thetadot*cos(phi)^3*cos(theta)*sin(phi) - 2*Iyy*K*l*omega2^2*cos(phi)*sin(phi)*sin(theta) + 2*Iyy*K*l*omega4^2*cos(phi)*sin(phi)*sin(theta) + 2*Izz*K*l*omega2^2*cos(phi)*sin(phi)*sin(theta) - 2*Izz*K*l*omega4^2*cos(phi)*sin(phi)*sin(theta) - 2*Ixx*Iyy*psidot*thetadot*sin(2*theta)*cos(phi)*sin(phi) + 2*Ixx*Izz*psidot*thetadot*sin(2*theta)*cos(phi)*sin(phi) - 2*Iyy*Izz*psidot*thetadot*sin(2*theta)*cos(phi)*sin(phi) + 2*Ixx*Iyy*psidot*thetadot*cos(phi)*cos(theta)*sin(phi)*sin(theta) - 2*Ixx*Izz*psidot*thetadot*cos(phi)*cos(theta)*sin(phi)*sin(theta) + 4*Iyy*Izz*psidot*thetadot*cos(phi)*cos(theta)*sin(phi)*sin(theta))/(2*cos(theta)*(- Iyy^2*cos(phi)^2*sin(phi)^2 - Iyy^2*sin(phi)^4 + Iyy^2*sin(phi)^2 + Izz*Iyy*cos(phi)^2*sin(phi)^2 + Izz*Iyy*cos(phi)^2 + Izz*Iyy*sin(phi)^4));
psi_ddot = (2*Iyy*b*omega1^2 - 2*Iyy*b*omega2^2 + 2*Iyy*b*omega3^2 - 2*Iyy*b*omega4^2 - Iyy^2*thetadot^2*sin(2*phi)*sin(theta) - 2*Iyy*b*omega1^2*sin(phi)^2 + 2*Iyy*b*omega2^2*sin(phi)^2 - 2*Iyy*b*omega3^2*sin(phi)^2 + 2*Iyy*b*omega4^2*sin(phi)^2 + 2*Izz*b*omega1^2*sin(phi)^2 - 2*Izz*b*omega2^2*sin(phi)^2 + 2*Izz*b*omega3^2*sin(phi)^2 - 2*Izz*b*omega4^2*sin(phi)^2 + 2*Iyy^2*psidot*thetadot*sin(2*theta) + 2*Iyy^2*phidot*thetadot*cos(theta) - 2*Iyy^2*phidot*thetadot*cos(theta)*sin(phi)^2 - 2*Izz^2*phidot*thetadot*cos(theta)*sin(phi)^2 - 2*Iyy*K*l*omega2^2*sin(theta) + 2*Iyy*K*l*omega4^2*sin(theta) - 2*Ixx*Iyy*psidot*thetadot*sin(2*theta) + Iyy^2*thetadot^2*sin(2*phi)*sin(phi)^2*sin(theta) + Izz^2*thetadot^2*sin(2*phi)*sin(phi)^2*sin(theta) - 2*Iyy^2*psidot*thetadot*sin(2*theta)*sin(phi)^2 + 2*Iyy^2*thetadot^2*cos(phi)*sin(phi)*sin(theta) - 2*Iyy^2*psidot*thetadot*cos(theta)*sin(theta) + 2*Ixx*Iyy*phidot*thetadot*cos(theta) - 2*Iyy*Izz*phidot*thetadot*cos(theta) - 2*Iyy^2*thetadot^2*cos(phi)*sin(phi)^3*sin(theta) - 2*Izz^2*thetadot^2*cos(phi)*sin(phi)^3*sin(theta) + Iyy*Izz*thetadot^2*sin(2*phi)*sin(theta) - 4*Iyy^2*phidot*thetadot*cos(phi)^2*cos(theta) - 2*Izz^2*psidot^2*cos(phi)*cos(theta)^2*sin(phi)^3*sin(theta) - 2*Izz^2*psidot^2*cos(phi)^3*cos(theta)^2*sin(phi)*sin(theta) - 2*Iyy*Izz*thetadot^2*sin(2*phi)*sin(phi)^2*sin(theta) + 2*Iyy^2*phidot*psidot*cos(phi)*cos(theta)^2*sin(phi)^3 + 2*Iyy^2*phidot*psidot*cos(phi)^3*cos(theta)^2*sin(phi) + 2*Izz^2*phidot*psidot*cos(phi)*cos(theta)^2*sin(phi)^3 + 2*Izz^2*phidot*psidot*cos(phi)^3*cos(theta)^2*sin(phi) + 4*Iyy^2*phidot*thetadot*cos(phi)^2*cos(theta)*sin(phi)^2 + 4*Izz^2*phidot*thetadot*cos(phi)^2*cos(theta)*sin(phi)^2 + 2*Iyy*K*l*omega2^2*sin(phi)^2*sin(theta) - 2*Iyy*K*l*omega4^2*sin(phi)^2*sin(theta) - 2*Izz*K*l*omega2^2*sin(phi)^2*sin(theta) + 2*Izz*K*l*omega4^2*sin(phi)^2*sin(theta) + 2*Ixx*Iyy*psidot*thetadot*sin(2*theta)*sin(phi)^2 - 2*Ixx*Izz*psidot*thetadot*sin(2*theta)*sin(phi)^2 + 2*Iyy*Izz*psidot*thetadot*sin(2*theta)*sin(phi)^2 - 2*Iyy*Izz*thetadot^2*cos(phi)*sin(phi)*sin(theta) + 2*Ixx*Iyy*psidot*thetadot*cos(theta)*sin(theta) + 2*Iyy*Izz*psidot*thetadot*cos(theta)*sin(theta) + 2*Iyy^2*psidot^2*cos(phi)*cos(theta)^2*sin(phi)*sin(theta) + 4*Iyy*Izz*thetadot^2*cos(phi)*sin(phi)^3*sin(theta) - 4*Iyy^2*phidot*psidot*cos(phi)*cos(theta)^2*sin(phi) + 4*Iyy*Izz*phidot*thetadot*cos(phi)^2*cos(theta) + 2*Iyy^2*psidot*thetadot*cos(theta)*sin(phi)^2*sin(theta) + 2*Izz^2*psidot*thetadot*cos(theta)*sin(phi)^2*sin(theta) - 2*Ixx*Iyy*phidot*thetadot*cos(theta)*sin(phi)^2 + 2*Ixx*Izz*phidot*thetadot*cos(theta)*sin(phi)^2 + 4*Iyy*Izz*phidot*thetadot*cos(theta)*sin(phi)^2 - 4*Iyy*Izz*phidot*psidot*cos(phi)*cos(theta)^2*sin(phi)^3 - 4*Iyy*Izz*phidot*psidot*cos(phi)^3*cos(theta)^2*sin(phi) - 8*Iyy*Izz*phidot*thetadot*cos(phi)^2*cos(theta)*sin(phi)^2 - Ixx*Iyy*psidot^2*sin(2*theta)*cos(phi)*cos(theta)*sin(phi) + Ixx*Izz*psidot^2*sin(2*theta)*cos(phi)*cos(theta)*sin(phi) - 2*Iyy*Izz*psidot^2*cos(phi)*cos(theta)^2*sin(phi)*sin(theta) + 2*Iyy*K*l*omega1^2*cos(phi)*cos(theta)*sin(phi) - 2*Iyy*K*l*omega3^2*cos(phi)*cos(theta)*sin(phi) - 2*Izz*K*l*omega1^2*cos(phi)*cos(theta)*sin(phi) + 2*Izz*K*l*omega3^2*cos(phi)*cos(theta)*sin(phi) - 2*Iyy^2*phidot*thetadot*sin(2*phi)*cos(phi)*cos(theta)*sin(phi) - 2*Izz^2*phidot*thetadot*sin(2*phi)*cos(phi)*cos(theta)*sin(phi) + 2*Ixx*Iyy*phidot*psidot*cos(phi)*cos(theta)^2*sin(phi) - 2*Ixx*Izz*phidot*psidot*cos(phi)*cos(theta)^2*sin(phi) + 4*Iyy*Izz*phidot*psidot*cos(phi)*cos(theta)^2*sin(phi) - 2*Ixx*Iyy*psidot*thetadot*cos(theta)*sin(phi)^2*sin(theta) + 2*Ixx*Izz*psidot*thetadot*cos(theta)*sin(phi)^2*sin(theta) - 4*Iyy*Izz*psidot*thetadot*cos(theta)*sin(phi)^2*sin(theta) + 2*Iyy*Izz*psidot^2*cos(phi)*cos(theta)^2*sin(phi)^3*sin(theta) + 2*Iyy*Izz*psidot^2*cos(phi)^3*cos(theta)^2*sin(phi)*sin(theta) + 4*Iyy*Izz*phidot*thetadot*sin(2*phi)*cos(phi)*cos(theta)*sin(phi))/(2*cos(theta)^2*(- Iyy^2*cos(phi)^2*sin(phi)^2 - Iyy^2*sin(phi)^4 + Iyy^2*sin(phi)^2 + Izz*Iyy*cos(phi)^2*sin(phi)^2 + Izz*Iyy*cos(phi)^2 + Izz*Iyy*sin(phi)^4));

if ((z_ddot<0 && z ==0) || z<0)
    rest=1;
    z_ddot=0;    
end

end

== matlab function cable_driven_parallel_robot2022/Actuators-CableTension-MovingPlatform/Moving Platform/Moving Platform/Moving Platform Transformation to Global ==
  settings: updateMethod=DISCRETE
  data: Vx input; Vy input; Vz input; roll input; pitch input; yaw input; Vbx output; Vby output; Vbz output; roll output; pitch output; yaw output; gx output; gy output; gz output; z input; rest output; Vx_min input; Vy_min input; Vz_min input; reste input
function [Vbx,Vby,Vbz,roll,pitch,yaw,gx,gy,gz,rest] = fcn(Vx,Vy,Vz,roll,pitch,yaw,z,Vx_min,Vy_min,Vz_min,reste)
rest=0;
V=[Vx;Vy;Vz];
G=[0;0;9.81];

R_x = [1    0       0; ...
       0  cos(roll) -sin(roll); ...
       0  sin(roll) cos(roll)];
   
R_y = [cos(pitch)  0   sin(pitch); ...
       0           1         0; ...
      -sin(pitch) 0   cos(pitch)]; 
   
R_z = [cos(yaw) -sin(yaw)  0; ...
       sin(yaw)  cos(yaw)  0; ...
       0           0       1]; 

BP_R_BN = R_z*R_y*R_x;

persistent R

if isempty(R)
R =   [1    0   0; ...
       0    1   0; ...
       0    0   1]; 
end

R = R*BP_R_BN;

Vel=R*V;

gcc=R'*G;

Vbx = Vel(1);

Vby = Vel(2);

Vbz = Vel(3);

if reste ==1
    Vbx = Vx_min;

    Vby = Vy_min;

    Vbz = Vz_min;
end

roll  = atan2(R(3,2),R(3,3));

pitch = atan2(-R(3,1),sqrt((R(1,1))^2+(R(1,2))^2));

yaw   = atan2(R(2,1),R(1,1));

gx= gcc(1);

gy= gcc(2);

gz= gcc(3);


if ((Vbz<0 && z ==0) || z<0)
    rest=1;
    Vbz=0;    
end

== matlab function cable_driven_parallel_robot2022/Actuators-CableTension-MovingPlatform/QuadRotor1/Subsystem/Subsystem/MATLAB Function ==
  data: rest0 input; rest output; init0 input; init output
function [rest,init] = fcn(rest0,init0)

if rest0==1
    rest=rest0;
    init=0;
else
  rest = rest0;
  init = init0;

end

== matlab function cable_driven_parallel_robot2022/Actuators-CableTension-MovingPlatform/QuadRotor1/Subsystem/Subsystem1/MATLAB Function ==
  data: rest0 input; rest output; init0 input; init output
function [rest,init] = fcn(rest0,init0)

if rest0==1
    rest=rest0;
    init=0;
else
  rest = rest0;
  init = init0;

end
